simulink model "LineFollowerTwin"  (R2025b)
settings: Solver=FixedStepDiscrete  StartTime=0.0  StopTime=cfg.stop_time  FixedStep=cfg.Ts  RelTol=1e-3
model workspace (MAT data in the model file):
  Kd = 0.03
  Ki = 0.015
  Kp = 0.45
  cfg.root = 'F:\DIGITAL TWEEN\line_follower_twin\full_project'
  cfg.trackMask = [0 0 0 0 0 0 0 0 0 0 0 0 ... (276271 elements, 431x641)]
  cfg.trackReflectance = [0 0 0 0 0 0 0 0 0 0 0 0 ... (276271 elements, 431x641)]
  cfg.map_width_m = 2.56
  cfg.map_height_m = 1.72
  cfg.meters_per_pixel_x = 0.004
  cfg.meters_per_pixel_y = 0.004
  cfg.line_width_m = 0.02
  cfg.stroke_width_px = 5
  cfg.referenceXY = [0.48 0.484 0.488 0.492 0.496 0.5 0.504 0.508 0.512 0.516 0.52 0.524 ... (6258 elements, 3129x2)]
  cfg.referenceArc = [0 0.004 0.008 0.012 0.016 0.02 0.024 0.028 0.032 0.036 0.04 0.044 ... (3129 elements, 1x3129)]
  cfg.x0 = 0.48
  cfg.y0 = 0.196
  cfg.theta0 = 0
  cfg.Ts = 0.02
  cfg.wheel_base_m = 0.12
  cfg.body_length_m = 0.16
  cfg.body_width_m = 0.1
  cfg.sensor_front_m = 0.05
  cfg.sensor_spacing_m = 0.008
  cfg.sensor_weights = [3.5 2.5 1.5 0.5 -0.5 -1.5 -2.5 -3.5]
  cfg.km = 0.35
  cfg.base_speed = 0.35
  cfg.Kp = 0.45
  cfg.Ki = 0.015
  cfg.Kd = 0.03
  cfg.integral_limit = 0.2
  cfg.anti_windup = 1
  cfg.derivative_tau = 0.08
  cfg.sensor_threshold = 0.5
  cfg.loss_timeout_s = 0.2
  cfg.stop_time = 100
  cfg.motor_left_factor = 1
  cfg.motor_right_factor = 1
  cfg.dropout_start_s = 1000
  cfg.dropout_duration_s = 0
  cfg.sensor_noise = 0
  cfg.environment_level = 0
  cfg.environment_seed = 7
  cfg.integration_method = 'exact_zoh'
  cfg.models_dir = 'F:\DIGITAL TWEEN\line_follower_twin\full_project\models'
  cfg.results_dir = 'F:\DIGITAL TWEEN\line_follower_twin\full_project\results'
  cfg.environment_input = [0 0.02 0.04 0.06 0.08 0.1 0.12 0.14 0.16 0.18 0.2 0.22 ... (65013 elements, 5001x13)]
  uL = 0.5
  uR = 0.5
undefined symbols (not defined in the file): DiscIntNeverNeededParam
settings Model: Creator=Xiaol  LastModifiedBy=Xiaol
settings DataIOCC: SaveOutput=off  SignalLogging=off

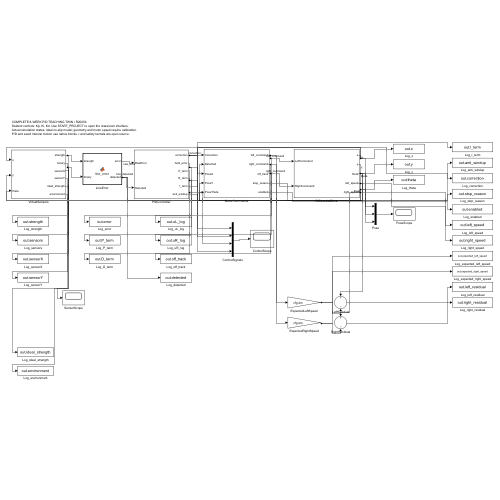
[thumbnail: Simulink's stored preview of the top-level diagram]
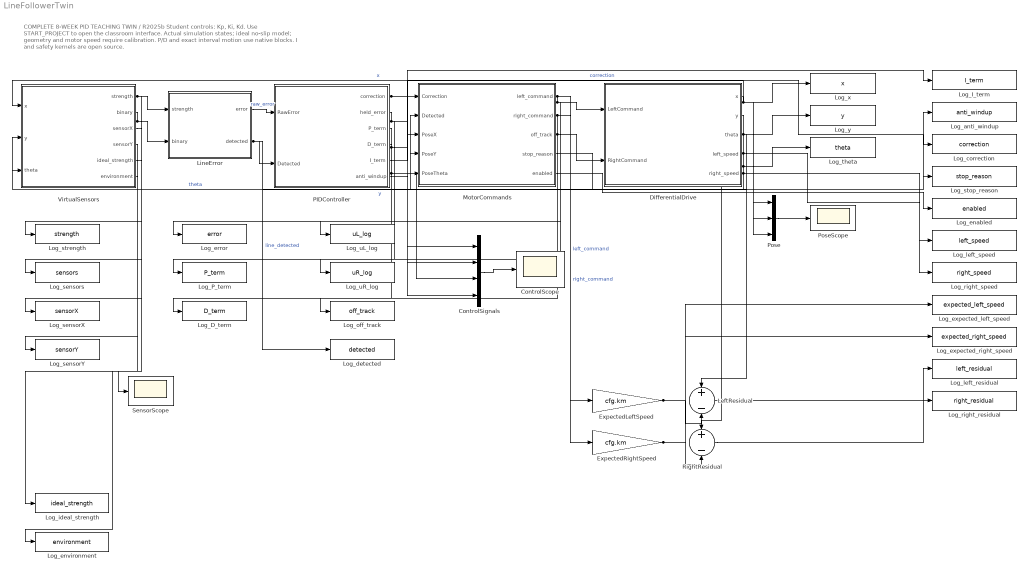
== system LineFollowerTwin ==
  note: COMPLETE 8-WEEK PID TEACHING TWIN / R2025b
      | Student controls: Kp, Ki, Kd. Use START_PROJECT to open the classroom interface.
      | Actual simulation states; ideal no-slip model; geometry and motor speed require calibration.
      | P/D and exact interval motion use native blocks. I and safety kernels are open source.
  ControlScope : Scope
  ControlSignals : Mux
  DifferentialDrive : Subsystem
  ExpectedLeftSpeed : Gain  Gain=cfg.km
  ExpectedRightSpeed : Gain  Gain=cfg.km
  LeftResidual : Sum  Inputs=+-
  LineError : MATLAB Function  TreatAsAtomicUnit=on
  Log_D_term : ToWorkspace  VariableName=D_term  SaveFormat=Timeseries  SampleTime=-1
  Log_I_term : ToWorkspace  VariableName=I_term  SaveFormat=Timeseries  SampleTime=-1
  Log_P_term : ToWorkspace  VariableName=P_term  SaveFormat=Timeseries  SampleTime=-1
  Log_anti_windup : ToWorkspace  VariableName=anti_windup  SaveFormat=Timeseries  SampleTime=-1
  Log_correction : ToWorkspace  VariableName=correction  SaveFormat=Timeseries  SampleTime=-1
  Log_detected : ToWorkspace  VariableName=detected  SaveFormat=Timeseries  SampleTime=-1
  Log_enabled : ToWorkspace  VariableName=enabled  SaveFormat=Timeseries  SampleTime=-1
  Log_environment : ToWorkspace  VariableName=environment  SaveFormat=Timeseries  SampleTime=-1
  Log_error : ToWorkspace  VariableName=error  SaveFormat=Timeseries  SampleTime=-1
  Log_expected_left_speed : ToWorkspace  VariableName=expected_left_speed  SaveFormat=Timeseries  SampleTime=-1
  Log_expected_right_speed : ToWorkspace  VariableName=expected_right_speed  SaveFormat=Timeseries  SampleTime=-1
  Log_ideal_strength : ToWorkspace  VariableName=ideal_strength  SaveFormat=Timeseries  SampleTime=-1
  Log_left_residual : ToWorkspace  VariableName=left_residual  SaveFormat=Timeseries  SampleTime=-1
  Log_left_speed : ToWorkspace  VariableName=left_speed  SaveFormat=Timeseries  SampleTime=-1
  Log_off_track : ToWorkspace  VariableName=off_track  SaveFormat=Timeseries  SampleTime=-1
  Log_right_residual : ToWorkspace  VariableName=right_residual  SaveFormat=Timeseries  SampleTime=-1
  Log_right_speed : ToWorkspace  VariableName=right_speed  SaveFormat=Timeseries  SampleTime=-1
  Log_sensorX : ToWorkspace  VariableName=sensorX  SaveFormat=Timeseries  SampleTime=-1
  Log_sensorY : ToWorkspace  VariableName=sensorY  SaveFormat=Timeseries  SampleTime=-1
  Log_sensors : ToWorkspace  VariableName=sensors  SaveFormat=Timeseries  SampleTime=-1
  Log_stop_reason : ToWorkspace  VariableName=stop_reason  SaveFormat=Timeseries  SampleTime=-1
  Log_strength : ToWorkspace  VariableName=strength  SaveFormat=Timeseries  SampleTime=-1
  Log_theta : ToWorkspace  VariableName=theta  SaveFormat=Timeseries  SampleTime=-1
  Log_uL_log : ToWorkspace  VariableName=uL_log  SaveFormat=Timeseries  SampleTime=-1
  Log_uR_log : ToWorkspace  VariableName=uR_log  SaveFormat=Timeseries  SampleTime=-1
  Log_x : ToWorkspace  VariableName=x  SaveFormat=Timeseries  SampleTime=-1
  Log_y : ToWorkspace  VariableName=y  SaveFormat=Timeseries  SampleTime=-1
  MotorCommands : Subsystem
  PIDController : Subsystem
  Pose : Mux  Inputs=3
  PoseScope : Scope
  RightResidual : Sum  Inputs=+-
  SensorScope : Scope
  VirtualSensors : Subsystem
  wires:
  DifferentialDrive/1(x) -> Log_x/1, Pose/1, VirtualSensors/1(x), MotorCommands/3(PoseX)  "x"
  DifferentialDrive/2(y) -> Log_y/1, Pose/2, VirtualSensors/2(y), MotorCommands/4(PoseY)  "y"
  DifferentialDrive/3(theta) -> Log_theta/1, Pose/3, VirtualSensors/3(theta), MotorCommands/5(PoseTheta)  "theta"
  Pose/1 -> PoseScope/1
  VirtualSensors/1(strength) -> LineError/1(strength), Log_strength/1
  VirtualSensors/2(binary) -> LineError/2(binary), Log_sensors/1, SensorScope/1
  LineError/1(error) -> PIDController/1(RawError)  "raw_error"
  LineError/2(detected) -> PIDController/2(Detected), MotorCommands/2(Detected), Log_detected/1  "line_detected"
  PIDController/1(correction) -> MotorCommands/1(Correction), ControlSignals/4, Log_correction/1  "correction"
  MotorCommands/1(left_command) -> DifferentialDrive/1(LeftCommand), Log_uL_log/1, ExpectedLeftSpeed/1  "left_command"
  MotorCommands/2(right_command) -> DifferentialDrive/2(RightCommand), Log_uR_log/1, ExpectedRightSpeed/1  "right_command"
  VirtualSensors/3(sensorX) -> Log_sensorX/1
  VirtualSensors/4(sensorY) -> Log_sensorY/1
  PIDController/2(held_error) -> Log_error/1, ControlSignals/1
  PIDController/3(P_term) -> Log_P_term/1, ControlSignals/2
  PIDController/4(D_term) -> Log_D_term/1, ControlSignals/3
  MotorCommands/3(off_track) -> Log_off_track/1
  ControlSignals/1 -> ControlScope/1
  VirtualSensors/5(ideal_strength) -> Log_ideal_strength/1
  VirtualSensors/6(environment) -> Log_environment/1
  DifferentialDrive/4(left_speed) -> LeftResidual/1, Log_left_speed/1
  ExpectedLeftSpeed/1 -> LeftResidual/2, Log_expected_left_speed/1
  DifferentialDrive/5(right_speed) -> RightResidual/1, Log_right_speed/1
  ExpectedRightSpeed/1 -> RightResidual/2, Log_expected_right_speed/1
  PIDController/5(I_term) -> Log_I_term/1
  PIDController/6(anti_windup) -> Log_anti_windup/1
  MotorCommands/4(stop_reason) -> Log_stop_reason/1
  MotorCommands/5(enabled) -> Log_enabled/1
  LeftResidual/1 -> Log_left_residual/1
  RightResidual/1 -> Log_right_residual/1

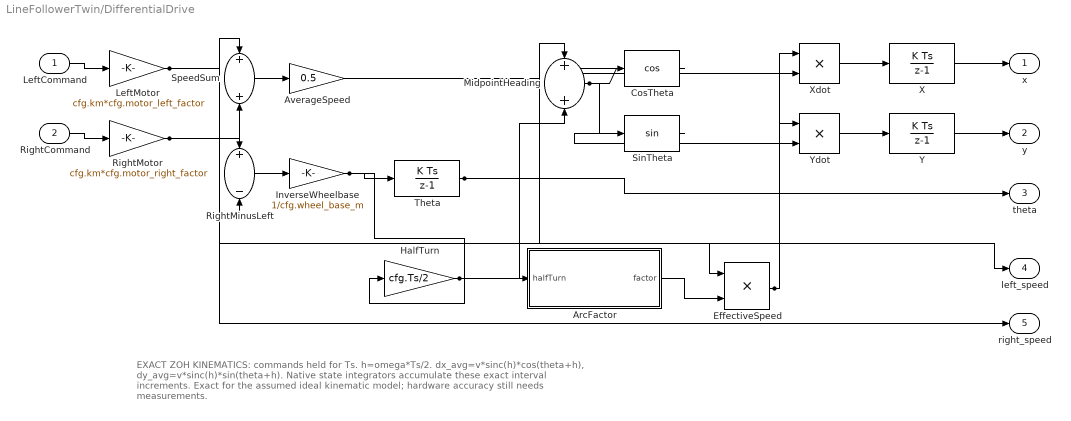
== system LineFollowerTwin/DifferentialDrive ==
  note: EXACT ZOH KINEMATICS: commands held for Ts. h=omega*Ts/2.
      | dx_avg=v*sinc(h)*cos(theta+h), dy_avg=v*sinc(h)*sin(theta+h).
      | Native state integrators accumulate these exact interval increments.
      | Exact for the assumed ideal kinematic model; hardware accuracy still needs measurements.
  LeftCommand : Inport
  RightCommand : Inport  Port=2
  ArcFactor : MATLAB Function  TreatAsAtomicUnit=on
  AverageSpeed : Gain  Gain=0.5
  CosTheta : Trigonometry  Operator=cos
  EffectiveSpeed : Product
  HalfTurn : Gain  Gain=cfg.Ts/2
  InverseWheelbase : Gain  Gain=1/cfg.wheel_base_m
  LeftMotor : Gain  Gain=cfg.km*cfg.motor_left_factor
  MidpointHeading : Sum
  RightMinusLeft : Sum  Inputs=+-
  RightMotor : Gain  Gain=cfg.km*cfg.motor_right_factor
  SinTheta : Trigonometry
  SpeedSum : Sum
  Theta : DiscreteIntegrator  gainval=1  InitialCondition=cfg.theta0  SampleTime=cfg.Ts  ICPrevOutput=DiscIntNeverNeededParam  ICPrevScaledInput=DiscIntNeverNeededParam
  X : DiscreteIntegrator  gainval=1  InitialCondition=cfg.x0  SampleTime=cfg.Ts  ICPrevOutput=DiscIntNeverNeededParam  ICPrevScaledInput=DiscIntNeverNeededParam
  Xdot : Product
  Y : DiscreteIntegrator  gainval=1  InitialCondition=cfg.y0  SampleTime=cfg.Ts  ICPrevOutput=DiscIntNeverNeededParam  ICPrevScaledInput=DiscIntNeverNeededParam
  Ydot : Product
  x : Outport
  y : Outport  Port=2
  theta : Outport  Port=3
  left_speed : Outport  Port=4
  right_speed : Outport  Port=5
  wires:
  LeftCommand/1 -> LeftMotor/1
  RightCommand/1 -> RightMotor/1
  LeftMotor/1 -> SpeedSum/1, RightMinusLeft/2, left_speed/1
  RightMotor/1 -> SpeedSum/2, RightMinusLeft/1, right_speed/1
  SpeedSum/1 -> AverageSpeed/1
  RightMinusLeft/1 -> InverseWheelbase/1
  InverseWheelbase/1 -> Theta/1, HalfTurn/1
  Theta/1 -> theta/1, MidpointHeading/1
  CosTheta/1 -> Xdot/2
  SinTheta/1 -> Ydot/2
  Xdot/1 -> X/1
  Ydot/1 -> Y/1
  X/1 -> x/1
  Y/1 -> y/1
  HalfTurn/1 -> MidpointHeading/2, ArcFactor/1(halfTurn)
  MidpointHeading/1 -> CosTheta/1, SinTheta/1
  AverageSpeed/1 -> EffectiveSpeed/1
  ArcFactor/1(factor) -> EffectiveSpeed/2
  EffectiveSpeed/1 -> Xdot/1, Ydot/1

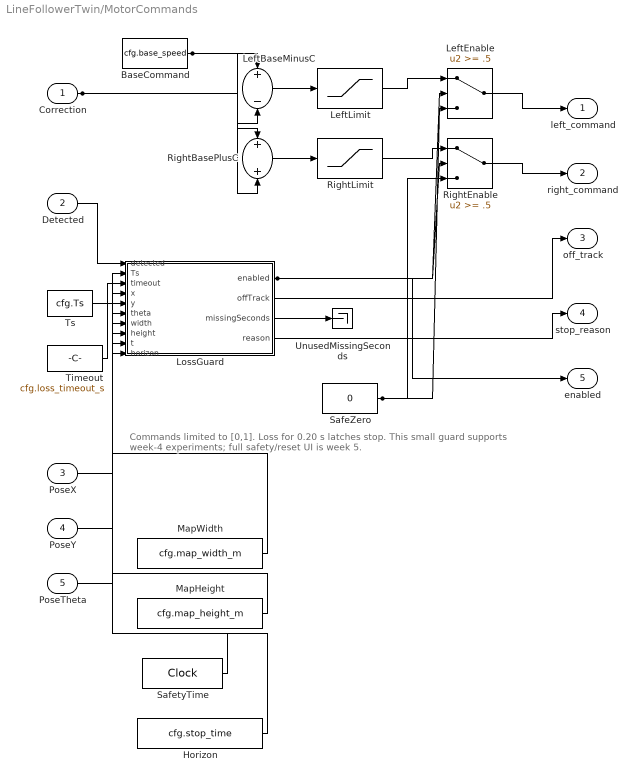
== system LineFollowerTwin/MotorCommands ==
  note: Commands limited to [0,1]. Loss for 0.20 s latches stop.
      | This small guard supports week-4 experiments; full safety/reset UI is week 5.
  Correction : Inport
  Detected : Inport  Port=2
  PoseX : Inport  Port=3
  PoseY : Inport  Port=4
  PoseTheta : Inport  Port=5
  BaseCommand : Constant  Value=cfg.base_speed  SampleTime=cfg.Ts
  Horizon : Constant  Value=cfg.stop_time
  LeftBaseMinusC : Sum  Inputs=+-
  LeftEnable : Switch  Threshold=.5  SaturateOnIntegerOverflow=off  InputSameDT=off
  LeftLimit : Saturate  UpperLimit=1  LowerLimit=0
  LossGuard : MATLAB Function  TreatAsAtomicUnit=on
  MapHeight : Constant  Value=cfg.map_height_m
  MapWidth : Constant  Value=cfg.map_width_m
  RightBasePlusC : Sum
  RightEnable : Switch  Threshold=.5  SaturateOnIntegerOverflow=off  InputSameDT=off
  RightLimit : Saturate  UpperLimit=1  LowerLimit=0
  SafeZero : Constant  Value=0
  SafetyTime : DigitalClock  SampleTime=cfg.Ts
  Timeout : Constant  Value=cfg.loss_timeout_s
  Ts : Constant  Value=cfg.Ts
  UnusedMissingSeconds : Terminator
  left_command : Outport
  right_command : Outport  Port=2
  off_track : Outport  Port=3
  stop_reason : Outport  Port=4
  enabled : Outport  Port=5
  wires:
  Detected/1 -> LossGuard/1(detected)
  Ts/1 -> LossGuard/2(Ts)
  Timeout/1 -> LossGuard/3(timeout)
  BaseCommand/1 -> LeftBaseMinusC/1, RightBasePlusC/1
  Correction/1 -> LeftBaseMinusC/2, RightBasePlusC/2
  LeftBaseMinusC/1 -> LeftLimit/1
  RightBasePlusC/1 -> RightLimit/1
  LossGuard/2(offTrack) -> off_track/1
  LossGuard/3(missingSeconds) -> UnusedMissingSeconds/1
  PoseX/1 -> LossGuard/4(x)
  PoseY/1 -> LossGuard/5(y)
  PoseTheta/1 -> LossGuard/6(theta)
  MapWidth/1 -> LossGuard/7(width)
  MapHeight/1 -> LossGuard/8(height)
  SafetyTime/1 -> LossGuard/9(t)
  Horizon/1 -> LossGuard/10(horizon)
  LeftLimit/1 -> LeftEnable/1
  LossGuard/1(enabled) -> LeftEnable/2, RightEnable/2, enabled/1
  SafeZero/1 -> LeftEnable/3, RightEnable/3
  LeftEnable/1 -> left_command/1
  RightLimit/1 -> RightEnable/1
  RightEnable/1 -> right_command/1
  LossGuard/4(reason) -> stop_reason/1

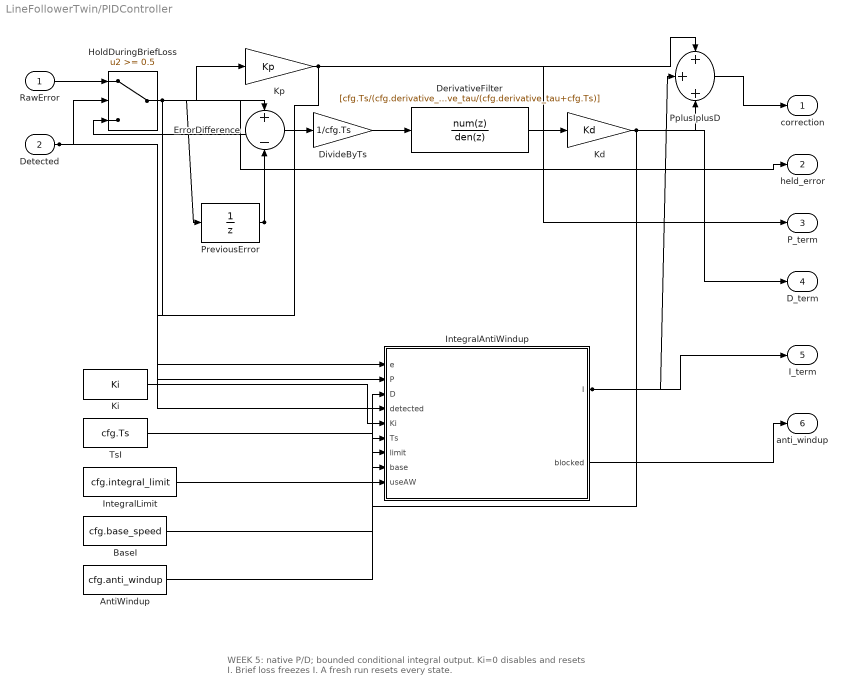
== system LineFollowerTwin/PIDController ==
  note: WEEK 5: native P/D; bounded conditional integral output.
      | Ki=0 disables and resets I. Brief loss freezes I. A fresh run resets every state.
  RawError : Inport
  Detected : Inport  Port=2
  AntiWindup : Constant  Value=cfg.anti_windup
  BaseI : Constant  Value=cfg.base_speed
  DerivativeFilter : DiscreteTransferFcn  Numerator=[cfg.Ts/(cfg.derivative_tau+cfg.Ts) 0]  Denominator=[1 -cfg.derivative_tau/(cfg.derivative_tau+cfg.Ts)]  SampleTime=cfg.Ts
  DivideByTs : Gain  Gain=1/cfg.Ts
  ErrorDifference : Sum  Inputs=+-
  HoldDuringBriefLoss : Switch  Threshold=0.5  SaturateOnIntegerOverflow=off  InputSameDT=off
  IntegralAntiWindup : MATLAB Function  TreatAsAtomicUnit=on
  IntegralLimit : Constant  Value=cfg.integral_limit
  Kd : Gain  Gain=Kd
  Ki : Constant  Value=Ki
  Kp : Gain  Gain=Kp
  PplusIplusD : Sum  Inputs=+++
  PreviousError : UnitDelay  SampleTime=cfg.Ts  HasFrameUpgradeWarning=on
  TsI : Constant  Value=cfg.Ts
  correction : Outport
  held_error : Outport  Port=2
  P_term : Outport  Port=3
  D_term : Outport  Port=4
  I_term : Outport  Port=5
  anti_windup : Outport  Port=6
  wires:
  RawError/1 -> HoldDuringBriefLoss/1
  Detected/1 -> HoldDuringBriefLoss/2, IntegralAntiWindup/4(detected)
  PreviousError/1 -> HoldDuringBriefLoss/3, ErrorDifference/2
  HoldDuringBriefLoss/1 -> PreviousError/1, Kp/1, ErrorDifference/1, held_error/1, IntegralAntiWindup/1(e)
  ErrorDifference/1 -> DivideByTs/1
  DivideByTs/1 -> DerivativeFilter/1
  DerivativeFilter/1 -> Kd/1
  Kp/1 -> P_term/1, IntegralAntiWindup/2(P), PplusIplusD/1
  Kd/1 -> D_term/1, IntegralAntiWindup/3(D), PplusIplusD/3
  PplusIplusD/1 -> correction/1
  Ki/1 -> IntegralAntiWindup/5(Ki)
  TsI/1 -> IntegralAntiWindup/6(Ts)
  IntegralLimit/1 -> IntegralAntiWindup/7(limit)
  BaseI/1 -> IntegralAntiWindup/8(base)
  AntiWindup/1 -> IntegralAntiWindup/9(useAW)
  IntegralAntiWindup/1(I) -> PplusIplusD/2, I_term/1
  IntegralAntiWindup/2(blocked) -> anti_windup/1

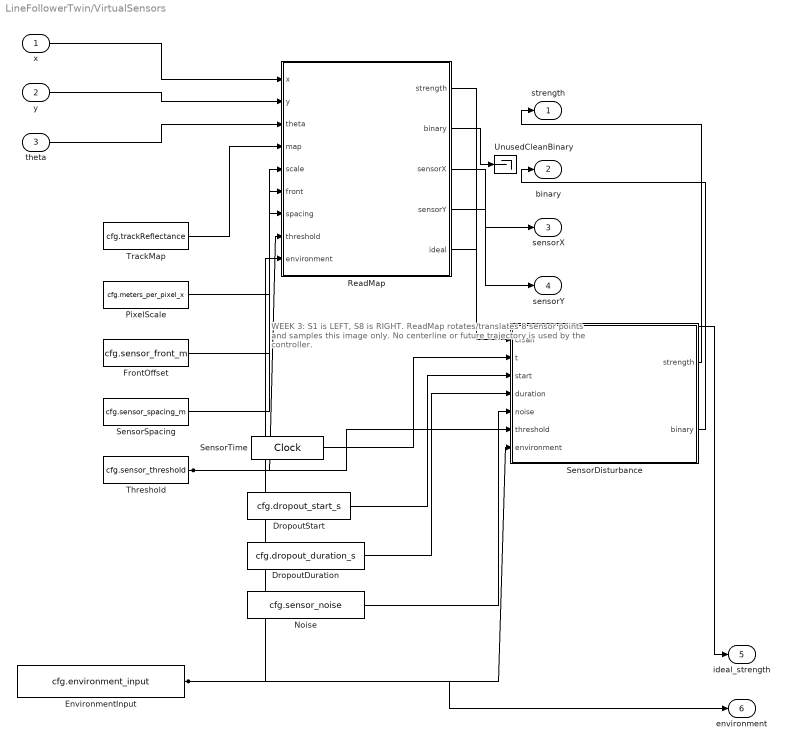
== system LineFollowerTwin/VirtualSensors ==
  note: WEEK 3: S1 is LEFT, S8 is RIGHT.
      | ReadMap rotates/translates 8 sensor points and samples this image only.
      | No centerline or future trajectory is used by the controller.
  x : Inport
  y : Inport  Port=2
  theta : Inport  Port=3
  DropoutDuration : Constant  Value=cfg.dropout_duration_s
  DropoutStart : Constant  Value=cfg.dropout_start_s
  EnvironmentInput : FromWorkspace  VariableName=cfg.environment_input  SampleTime=cfg.Ts  Interpolate=off  OutputAfterFinalValue=Holding final value
  FrontOffset : Constant  Value=cfg.sensor_front_m
  Noise : Constant  Value=cfg.sensor_noise
  PixelScale : Constant  Value=cfg.meters_per_pixel_x
  ReadMap : MATLAB Function  TreatAsAtomicUnit=on
  SensorDisturbance : MATLAB Function  TreatAsAtomicUnit=on
  SensorSpacing : Constant  Value=cfg.sensor_spacing_m
  SensorTime : DigitalClock  SampleTime=cfg.Ts
  Threshold : Constant  Value=cfg.sensor_threshold
  TrackMap : Constant  Value=cfg.trackReflectance
  UnusedCleanBinary : Terminator
  strength : Outport
  binary : Outport  Port=2
  sensorX : Outport  Port=3
  sensorY : Outport  Port=4
  ideal_strength : Outport  Port=5
  environment : Outport  Port=6
  wires:
  x/1 -> ReadMap/1(x)
  y/1 -> ReadMap/2(y)
  theta/1 -> ReadMap/3(theta)
  TrackMap/1 -> ReadMap/4(map)
  PixelScale/1 -> ReadMap/5(scale)
  FrontOffset/1 -> ReadMap/6(front)
  SensorSpacing/1 -> ReadMap/7(spacing)
  Threshold/1 -> ReadMap/8(threshold), SensorDisturbance/6(threshold)
  ReadMap/3(sensorX) -> sensorX/1
  ReadMap/4(sensorY) -> sensorY/1
  EnvironmentInput/1 -> ReadMap/9(environment), environment/1, SensorDisturbance/7(environment)
  ReadMap/5(ideal) -> ideal_strength/1
  ReadMap/1(strength) -> SensorDisturbance/1(clean)
  SensorTime/1 -> SensorDisturbance/2(t)
  DropoutStart/1 -> SensorDisturbance/3(start)
  DropoutDuration/1 -> SensorDisturbance/4(duration)
  Noise/1 -> SensorDisturbance/5(noise)
  SensorDisturbance/1(strength) -> strength/1
  SensorDisturbance/2(binary) -> binary/1
  ReadMap/2(binary) -> UnusedCleanBinary/1

== matlab function LineFollowerTwin/LineError ==
  data: strength input; error output; binary input; detected output
function [error,detected] = line_error(strength,binary)
%#codegen
% Positive error: black line is on the LEFT, so increase right-side speed.
detected=double(any(binary>0.5));
error=0;
if detected
    total=0; weighted=0;
    for i=1:8
        total=total+strength(i);
        weighted=weighted+strength(i)*(4.5-i);
    end
    error=weighted/(3.5*max(total,1e-12));
end
end

== matlab function LineFollowerTwin/VirtualSensors/ReadMap ==
  data: x input; strength output; y input; theta input; map input; scale input; front input; spacing input; threshold input; binary output; sensorX output; sensorY output; environment input; ideal output
function [strength,binary,sensorX,sensorY,ideal] = virtual_sensors(x,y,theta,map,scale,front,spacing,threshold,environment)
%#codegen
% S1..S8 run LEFT to RIGHT as seen looking forward. Outside-map values are zero.
strength=zeros(1,8); binary=zeros(1,8);ideal=zeros(1,8);
sensorX=zeros(1,8); sensorY=zeros(1,8);
ct=cos(theta); st=sin(theta);
for i=1:8
    localY=(4.5-i)*spacing;
    nominalX=x+ct*front-st*localY;
    nominalY=y+st*front+ct*localY;
    ideal(i)=sample_map(map,scale,nominalX,nominalY);
    X=nominalX+ct*environment(3)-st*environment(4);
    Y=nominalY+st*environment(3)+ct*environment(4);
    sensorX(i)=X; sensorY(i)=Y;
    strength(i)=sample_map(map,scale,X,Y);
    binary(i)=double(strength(i)>=threshold);
end
end
function value=sample_map(map,scale,X,Y)
[H,W]=size(map);col=1+X/scale;row=H-Y/scale;value=0;
if col>=1 && col<=W && row>=1 && row<=H
    c0=floor(col);r0=floor(row);c1=min(c0+1,W);r1=min(r0+1,H);
    dc=col-c0;dr=row-r0;
    value=(1-dr)*((1-dc)*map(r0,c0)+dc*map(r0,c1)) ...
        +dr*((1-dc)*map(r1,c0)+dc*map(r1,c1));
end
end

== matlab function LineFollowerTwin/MotorCommands/LossGuard ==
  data: detected input; enabled output; Ts input; timeout input; offTrack output; missingSeconds output; x input; y input; theta input; width input; height input; t input; horizon input; reason output
function [enabled,offTrack,missingSeconds,reason]=full_guard(detected,Ts,timeout,x,y,theta,width,height,t,horizon)
%#codegen
% Latched stop reason: 0 run, 1 lost line, 2 out of bounds, 3 numeric, 4 timeout.
persistent elapsed active stopped code
if isempty(elapsed),elapsed=0;active=false;stopped=false;code=0;end
if detected,elapsed=0;active=false;elseif active,elapsed=elapsed+Ts;else,elapsed=0;active=true;end
if ~stopped
    if ~isfinite(x) || ~isfinite(y) || ~isfinite(theta),code=3;
    elseif x<0 || y<0 || x>width || y>height,code=2;
    elseif elapsed>=timeout-1e-12,code=1;
    elseif t>=horizon-1e-12,code=4;
    end
    stopped=code~=0;
end
enabled=double(~stopped);offTrack=double(code==1);missingSeconds=elapsed;reason=code;
end

== matlab function LineFollowerTwin/DifferentialDrive/ArcFactor ==
  data: halfTurn input; factor output
function factor = arc_factor(halfTurn)
%#codegen
% sin(h)/h; exact displacement factor for constant twist over one sample.
if abs(halfTurn)<1e-4
    h2=halfTurn*halfTurn;
    factor=1-h2/6+h2*h2/120;
else
    factor=sin(halfTurn)/halfTurn;
end
end

== matlab function LineFollowerTwin/PIDController/IntegralAntiWindup ==
  data: e input; I output; P input; D input; detected input; Ki input; Ts input; limit input; base input; useAW input; blocked output
function [I,blocked]=integral_aw(e,P,D,detected,Ki,Ts,limit,base,useAW)
%#codegen
% Bounded integral OUTPUT. Conditional integration uses downstream motor limits.
persistent state
if isempty(state),state=0;end
blocked=0;
if Ki==0,state=0;elseif detected
    delta=Ki*e*Ts;
    candidate=min(max(state+delta,-limit),limit);
    total=P+D+candidate;
    authority=min(base,1-base); % either wheel saturates beyond this correction
    if useAW && abs(total)>authority && total*delta>0
        blocked=1;
    else
        state=candidate;
    end
end
I=state;
end

== matlab function LineFollowerTwin/VirtualSensors/SensorDisturbance ==
  data: clean input; strength output; t input; start input; duration input; noise input; threshold input; environment input; binary output
function [strength,binary]=sensor_fault(clean,t,start,duration,noise,threshold,environment)
%#codegen
% Optical errors affect the observed strengths before thresholding and control.
strength=zeros(1,8);binary=zeros(1,8);
for k=1:8
    value=environment(1)*clean(k)+environment(2)+environment(k+4) ...
        +noise*sin(2*pi*(7+k)*t+.37*k);
    strength(k)=min(max(value,0),1);
    if t>=start-1e-12 && t<start+duration-1e-12,strength(k)=0;end
    binary(k)=double(strength(k)>=threshold);
end
end
